simulink model "Active_Power_Filter"  (R2023b)
settings: Solver=VariableStepAuto  StartTime=0.0  StopTime=0.5  RelTol=1e-3
libraries: spsSeriesRLCBranchLib x5, spsCurrentMeasurementLib x2, spsUniversalBridgeLib x2, spsVoltageMeasurementLib x2, spsACVoltageSourceLib x1, spsMeanLib x1, slpidlib x1, powerlib_extras x1, spsTHDLib x1, spspowerguiLib x1, simulink x1
settings Model: SimulationMode=accelerator  Creator=abc6820292  LastModifiedBy=Qu
settings DataIOCC: ReturnWorkspaceOutputs=off
settings DebuggingCC: UnconnectedInputMsg=warning  UnconnectedOutputMsg=warning  UnconnectedLineMsg=warning
settings ModelReferenceCC: EnableRefExpFcnMdlSchedulingChecks=on
settings RTWCC: DLArmComputeVersion=19.05

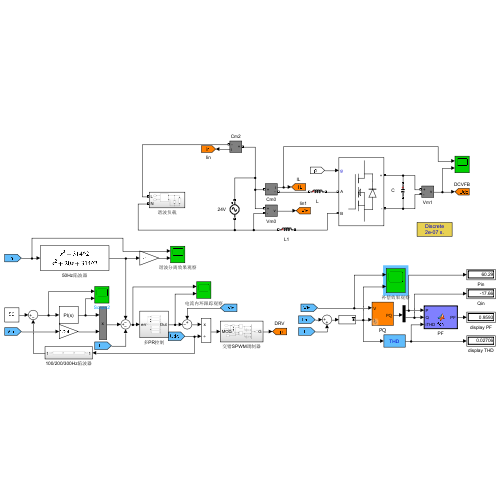
[thumbnail: Simulink's stored preview of the top-level diagram]
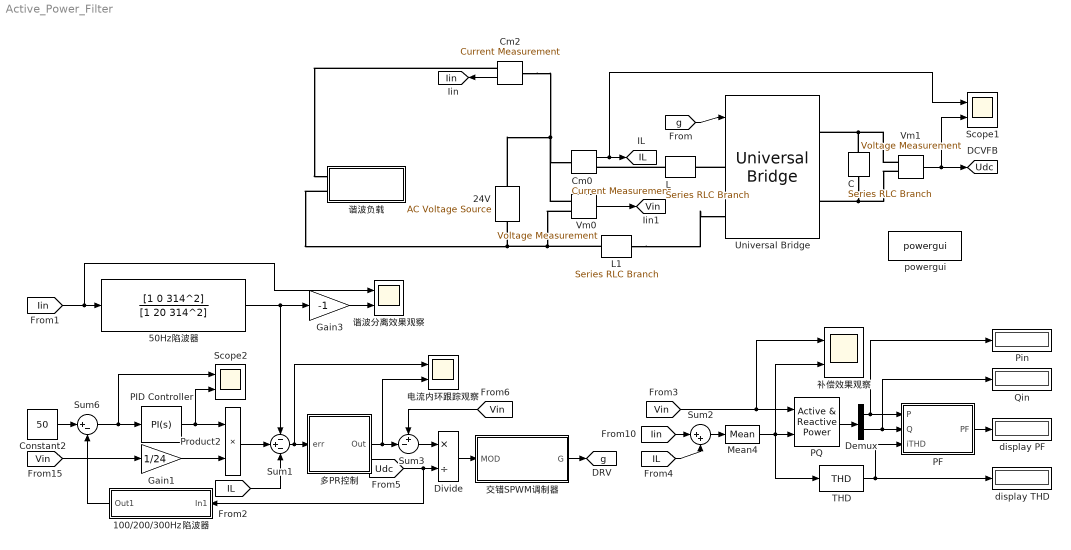
== system Active_Power_Filter ==
  100/200/300Hz陷波器 : Subsystem
  24V : spsACVoltageSourceLib/AC Voltage Source  Amplitude=24*1.414  Phase=0  Frequency=50  SampleTime=0  Measurements=None  BusType=swing  Pref=10e3  Qref=0  Qmin=-inf  Qmax=+inf
  50Hz陷波器 : TransferFcn  Numerator=[1 0 314^2]  Denominator=[1 20 314^2]
  C : spsSeriesRLCBranchLib/Series RLC Branch  LConnTagsString=__new0  RConnTagsString=__new0  BranchType=C  Resistance=0.01  Inductance=7e-4  SetiL0=off  InitialCurrent=0  Capacitance=4e-3  Setx0=on  InitialVoltage=50  Measurements=None
  Cm0 : spsCurrentMeasurementLib/Current Measurement  PhasorSimulation=off  OutputType=Complex  PSBequivalent=0
  Cm2 : spsCurrentMeasurementLib/Current Measurement  PhasorSimulation=off  OutputType=Complex  PSBequivalent=0
  Constant2 : Constant  Value=50
  Demux : Demux  Outputs=2
  Divide : Product  Inputs=*/
  Gain1 : Gain  Gain=1/24
  Gain3 : Gain  Gain=-1
  L : spsSeriesRLCBranchLib/Series RLC Branch  LConnTagsString=__new0  RConnTagsString=__new0  BranchType=L  Resistance=0.05  Inductance=1e-4  SetiL0=off  InitialCurrent=0  Capacitance=1e-3  Setx0=off  InitialVoltage=0  Measurements=None
  L1 : spsSeriesRLCBranchLib/Series RLC Branch  LConnTagsString=__new0  RConnTagsString=__new0  BranchType=L  Resistance=0.05  Inductance=1e-4  SetiL0=off  InitialCurrent=0  Capacitance=1e-3  Setx0=off  InitialVoltage=0  Measurements=None
  Mean4 : spsMeanLib/Mean  Freq=25000  Vinit=0  Ts=0
  PF : MATLAB Function  TreatAsAtomicUnit=on
  PID Controller : slpidlib/PID Controller  Controller=PI  Form=Parallel  TimeDomain=Continuous-time  UseExternalTs=off  SampleTime=-1  IntegratorMethod=Forward Euler  FilterMethod=Forward Euler  ControllerParametersSource=internal  P=0.4  I=5  UseKiTs=off  D=0.005  N=100  UseFilter=on  TunerSelectOption=Transfer Function Based (PID Tuner App)  InitialConditionSource=internal  InitialConditionForIntegrator=0  InitialConditionForFilter=0  DifferentiatorICPrevScaledInput=0  ExternalReset=none  TrackingMode=off  Kt=1  LimitOutput=off  SatLimitsSource=internal  UpperSaturationLimit=200  LowerSaturationLimit=0  LinearizeAsGain=on  AntiWindupMode=clamping  Kb=1  LimitIntegrator=off  UpperIntegratorSaturationLimit=inf  LowerIntegratorSaturationLimit=-inf  POutMin=[]  POutMax=[]  IOutMin=[]  IOutMax=[]  DOutMin=[]  DOutMax=[]  NOutMin=[]  NOutMax=[]  SumOutMin=[]  SumOutMax=[]  SaturationOutMin=[]  SaturationOutMax=[]  PParamMin=[]  PParamMax=[]  IParamMin=[]  IParamMax=[]  DParamMin=[]  DParamMax=[]  NParamMin=[]  NParamMax=[]  KbParamMin=[]  KbParamMax=[]  KtParamMin=[]  KtParamMax=[]  KbOutMin=[]  KbOutMax=[]  KtOutMin=[]  KtOutMax=[]  IntegratorOutMin=[]  IntegratorOutMax=[]  FilterOutMin=[]  FilterOutMax=[]  SumI1OutMin=[]  SumI1OutMax=[]  SumI2OutMin=[]  SumI2OutMax=[]  SumI3OutMin=[]  SumI3OutMax=[]  SumI4OutMin=[]  SumI4OutMax=[]  SumDOutMin=[]  SumDOutMax=[]  DifferentiatorOutMin=[]  DifferentiatorOutMax=[]  FilterDiffOutCoefMin=[]  FilterDiffOutCoefMax=[]  ReciprocalOutMin=[]  ReciprocalOutMax=[]  SumDenOutMin=[]  SumDenOutMax=[]  SumNumOutMin=[]  SumNumOutMax=[]  DivideOutMin=[]  DivideOutMax=[]  UdiffTsProdOutMin=[]  UdiffTsProdOutMax=[]  NTsProdOutMin=[]  NTsProdOutMax=[]  UintegralTsProdOutMin=[]  UintegralTsProdOutMax=[]  UngainTsProdOutMin=[]  UngainTsProdOutMax=[]  ClampingZeroOutDataTypeStr=Inherit: Inherit via back propagation  ClampingZeroOutMin=[]  ClampingZeroOutMax=[]  FilterDenConstantOutDataTypeStr=Inherit: Inherit via back propagation  FilterDenConstantOutMin=[]  FilterDenConstantOutMax=[]  PCopyOutDataTypeStr=Inherit: Inherit via back propagation  PCopyOutMin=[]  PCopyOutMax=[]  NCopyOutDataTypeStr=Inherit: Inherit via back propagation  NCopyOutMin=[]  NCopyOutMax=[]  IntegratorContinuousStateAttributes=''  IntegratorStateMustResolveToSignalObject=off  IntegratorRTWStateStorageClass=Auto  FilterContinuousStateAttributes=''  FilterStateMustResolveToSignalObject=off  FilterRTWStateStorageClass=Auto  ParallelPVariant=InternalParameters  IdealPVariant=Disabled  IVariant=InternalParameters  DVariant=Disabled  IntegratorVariant=Continuous  SatVariant=Disabled  AWVariant=Passthrough  PCopyVariant=Disabled  TRVariant=Disabled  FdbkBlocksVariant=Forward  IdealPFdbkVariant=Disabled  SatFdbkVariant=Disabled  DerivativeFilterVariant=Disabled  NVariant=Disabled  NCopyVariant=Disabled_SignalSpec  FilterICVariant=Disabled  IntegratorICVariant=InternalICs  ExternalResetVariant=Disabled  TRSumVariant=Passthrough  SumFdbkVariant=Disabled  SumVariant=Sum_PI  TsampFilterVariant=InternalTs  TsampNgainVariant=Passthrough  TsampIntegralVariant=Disabled_SignalSpec  ExternalSaturationOutDataTypeStr=Inherit: Same as second input
  PQ : powerlib_extras/Measurements/Active & Reactive Power  f1=50
  Pin : Display
      settings: Format=bank
  Product2 : Product  RndMeth=Zero
  Qin : Display
  Scope1 : Scope  NumInputPorts=2
  Scope2 : Scope  NumInputPorts=2
  Sum1 : Sum  Inputs=-+-
  Sum2 : Sum  Inputs=|++
  Sum3 : Sum  Inputs=+-|
  Sum6 : Sum  Inputs=|+-
  THD : spsTHDLib/THD  Freq=50  Ts=0
  Universal Bridge : spsUniversalBridgeLib/Universal Bridge  Arms=2  SnubberResistance=1e5  SnubberCapacitance=1e-9  Device=MOSFET / Diodes  Ron=1e-2  Lon=0  ForwardVoltages="[  1  1  ]"  ForwardVoltage=0  GTOparameters=[ 10e-6 , 20e-6 ]  IGBTparameters=[ 1e-6 , 2e-6 ]  Measurements=None  Measurements_2=None  converterType=Rectifier
  Vm0 : spsVoltageMeasurementLib/Voltage Measurement  PhasorSimulation=off  OutputType=Complex  PSBequivalent=0
  Vm1 : spsVoltageMeasurementLib/Voltage Measurement  PhasorSimulation=off  OutputType=Complex  PSBequivalent=0
  display PF : Display
  display THD : Display
  powergui : spspowerguiLib/powergui  SimulationMode=Discrete  SampleTime=2e-7  frequency=60  Iterations=50  frequencyindice=0  Pbase=100e6  ErrMax=1e-4  UnitsV=kV  UnitsW=MW  buscounter=0  FunctionMessages=off  echomessages=off  EnableUseOfTLC=off  CurrentSourceSwitches=off  DisableSnubberDevices=off  DisableRonSwitches=off  DisableVfSwitches=off  DisplayEquations=off  AutomaticDiscreteSolvers=off  SolverType=Tustin/Backward Euler (TBE)  Interpol=off  ExternalGateDelay=off  methode=off  Ts=0  x0status=blocks  SPID=off  SwTol=0  HookPort=off  NonlinearTolerance=1e-4  nMaxIteration=100  ContinueOnMaxIteration=off  RestoreLinks=warning  ResistiveCurrentMeasurement=off  Frange=[0:2:500]  Ylog=off  Xlog=on  ShowGrid=off  save=off  variable=ZData  structure=QQQQQ  ZoomFFT=off  StartTime=0.5  cycles=15  DisplayStyle=1  fundamental=50  FreqAxis=off  MaxFrequency=1000  frequencyindicesteady=1  RmsSteady=1  display=off
  交错SPWM调制器 : Subsystem
  多PR控制 : Subsystem
  电流内环跟踪观察 : Scope  NumInputPorts=2
  补偿效果观察 : Scope  NumInputPorts=2
  谐波分离效果观察 : Scope  NumInputPorts=2
  谐波负载 : Subsystem
  tag scope: IL=global, Iin=global, Udc=global, Vin=global, g=global
  wires:
  Cm0/1 -> Scope1/1, [IL]
  Vm0/1 -> [Vin]
  Demux/1 -> Pin/1, PF/1(P)
  Demux/2 -> Qin/1, PF/2(Q)
  PF/1(PF) -> display PF/1
  PQ/1 -> Demux/1
  THD/1 -> display THD/1, PF/3(iTHD)
  [Vin] -> 补偿效果观察/1, PQ/1
  Mean4/1 -> THD/1, 补偿效果观察/2, PQ/2
  Vm1/1 -> Scope1/2, [Udc]
  PID Controller/1 -> Scope2/2, Product2/1
  Gain1/1 -> Product2/2
  Sum6/1 -> Scope2/1, PID Controller/1
  [Vin] -> Gain1/1
  [g] -> Universal Bridge/1
  交错SPWM调制器/1(G) -> [g]
  Sum1/1 -> 电流内环跟踪观察/1, 多PR控制/1(err)
  Sum3/1 -> Divide/1
  多PR控制/1(Out) -> 电流内环跟踪观察/2, Sum3/2
  Divide/1 -> 交错SPWM调制器/1(MOD)
  [Udc] -> 100/200/300Hz陷波器/1(In1), Divide/2
  [Vin] -> Sum3/1
  [IL] -> Sum1/3
  [Iin] -> Sum2/1
  [IL] -> Sum2/2
  Sum2/1 -> Mean4/1
  Cm2/1 -> [Iin]
  50Hz陷波器/1 -> Gain3/1, Sum1/1
  [Iin] -> 谐波分离效果观察/1, 50Hz陷波器/1
  Product2/1 -> Sum1/2
  Constant2/1 -> Sum6/1
  Gain3/1 -> 谐波分离效果观察/2
  100/200/300Hz陷波器/1(Out1) -> Sum6/2
  connections:
  Vm1/LConn1 -- Universal Bridge/RConn1 -- C/LConn1
  24V/RConn1 -- Cm2/LConn1 -- Vm0/LConn1 -- Cm0/LConn1
  Vm0/LConn2 -- L1/LConn1 -- 谐波负载/LConn2 -- 24V/LConn1
  L/LConn1 -- Cm0/RConn1
  Universal Bridge/LConn1 -- L/RConn1
  L1/RConn1 -- Universal Bridge/LConn2
  Cm2/RConn1 -- 谐波负载/LConn1
  Vm1/LConn2 -- C/RConn1 -- Universal Bridge/RConn2

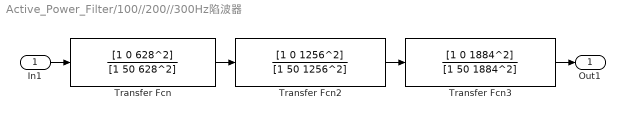
== system Active_Power_Filter/100//200//300Hz陷波器 ==
  In1 : Inport
  Transfer Fcn : TransferFcn  Numerator=[1 0 628^2]  Denominator=[1 50 628^2]
  Transfer Fcn2 : TransferFcn  Numerator=[1 0 1256^2]  Denominator=[1 50 1256^2]
  Transfer Fcn3 : TransferFcn  Numerator=[1 0 1884^2]  Denominator=[1 50 1884^2]
  Out1 : Outport
  wires:
  Transfer Fcn2/1 -> Transfer Fcn3/1
  In1/1 -> Transfer Fcn/1
  Transfer Fcn/1 -> Transfer Fcn2/1
  Transfer Fcn3/1 -> Out1/1

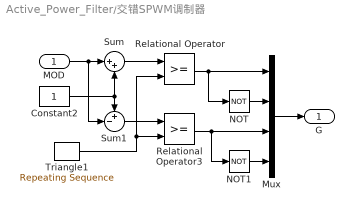
== system Active_Power_Filter/交错SPWM调制器 ==
  MOD : Inport
  Constant2 : Constant
  Mux : Mux
  NOT : Logic  Operator=NOT  IconShape=distinctive  AllPortsSameDT=off  OutDataTypeStr=boolean
  NOT1 : Logic  Operator=NOT  IconShape=distinctive  AllPortsSameDT=off  OutDataTypeStr=boolean
  Relational Operator : RelationalOperator  OutDataTypeStr=boolean  InputSameDT=off
  Relational Operator3 : RelationalOperator  OutDataTypeStr=boolean  InputSameDT=off
  Sum : Sum  Inputs=|++
  Sum1 : Sum  Inputs=+-|
  Triangle1 : simulink/Sources/Repeating Sequence  rep_seq_t=[0 1/50000/2 1/50000]  rep_seq_y=[0 1 0]
  G : Outport
  wires:
  MOD/1 -> Sum1/2, Sum/1
  Triangle1/1 -> Relational Operator/2, Relational Operator3/2
  Mux/1 -> G/1
  Relational Operator/1 -> NOT/1, Mux/1
  Relational Operator3/1 -> NOT1/1, Mux/3
  NOT/1 -> Mux/2
  NOT1/1 -> Mux/4
  Sum/1 -> Relational Operator/1
  Sum1/1 -> Relational Operator3/1
  Constant2/1 -> Sum/2, Sum1/1

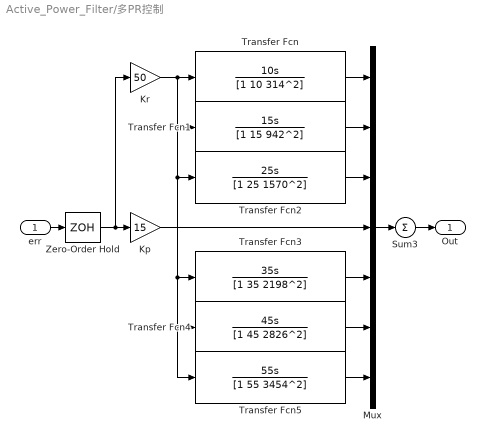
== system Active_Power_Filter/多PR控制 ==
  err : Inport
  Kp : Gain  Gain=15
  Kr : Gain  Gain=50
  Mux : Mux  Inputs=7
  Sum3 : Sum  Inputs=+
  Transfer Fcn : TransferFcn  Numerator=[10 0]  Denominator=[1 10 314^2]
  Transfer Fcn1 : TransferFcn  Numerator=[15 0]  Denominator=[1 15 942^2]
  Transfer Fcn2 : TransferFcn  Numerator=[25 0]  Denominator=[1 25 1570^2]
  Transfer Fcn3 : TransferFcn  Numerator=[35 0]  Denominator=[1 35 2198^2]
  Transfer Fcn4 : TransferFcn  Numerator=[45 0]  Denominator=[1 45 2826^2]
  Transfer Fcn5 : TransferFcn  Numerator=[55 0]  Denominator=[1 55 3454^2]
  Zero-Order Hold : ZeroOrderHold  SampleTime=1/100000
  Out : Outport
  wires:
  Transfer Fcn1/1 -> Mux/2
  Transfer Fcn2/1 -> Mux/3
  Transfer Fcn4/1 -> Mux/6
  Transfer Fcn5/1 -> Mux/7
  Kr/1 -> Transfer Fcn5/1, Transfer Fcn4/1, Transfer Fcn3/1, Transfer Fcn2/1, Transfer Fcn1/1, Transfer Fcn/1
  Transfer Fcn/1 -> Mux/1
  Mux/1 -> Sum3/1
  Sum3/1 -> Out/1
  Zero-Order Hold/1 -> Kr/1, Kp/1
  err/1 -> Zero-Order Hold/1
  Transfer Fcn3/1 -> Mux/5
  Kp/1 -> Mux/4

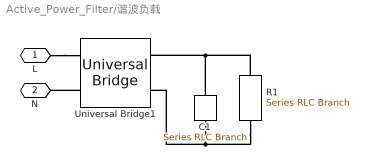
== system Active_Power_Filter/谐波负载 ==
  C1 : spsSeriesRLCBranchLib/Series RLC Branch  LConnTagsString=__new0  RConnTagsString=__new0  BranchType=C  Resistance=0.01  Inductance=7e-4  SetiL0=off  InitialCurrent=0  Capacitance=2e-3  Setx0=on  InitialVoltage=42  Measurements=None
  R1 : spsSeriesRLCBranchLib/Series RLC Branch  LConnTagsString=__new0  RConnTagsString=__new0  BranchType=R  Resistance=15  Inductance=7e-4  SetiL0=off  InitialCurrent=0  Capacitance=1e-3  Setx0=off  InitialVoltage=0  Measurements=None
  Universal Bridge1 : spsUniversalBridgeLib/Universal Bridge  Arms=2  SnubberResistance=1e5  SnubberCapacitance=1e-9  Device=Diodes  Ron=0.1  Lon=0  ForwardVoltages="[  1  1  ]"  ForwardVoltage=0.7  GTOparameters=[ 10e-6 , 20e-6 ]  IGBTparameters=[ 1e-6 , 2e-6 ]  Measurements=None  Measurements_2=None  converterType=Rectifier
  L : PMIOPort  Side=Left
  N : PMIOPort  Port=2  Side=Left
  connections:
  Universal Bridge1/LConn2 -- N/RConn1
  L/RConn1 -- Universal Bridge1/LConn1
  C1/LConn1 -- Universal Bridge1/RConn1 -- R1/LConn1
  C1/RConn1 -- Universal Bridge1/RConn2 -- R1/RConn1

== matlab function Active_Power_Filter/PF ==
  data: P input; PF output; Q input; iTHD input
function PF = fcn(P,Q,iTHD)
% This block supports an embeddable subset of the MATLAB language.
% See the help menu for details. 
PF=(P/sqrt(P*P+Q*Q))/(sqrt(1+iTHD*iTHD));
